simulink model "IEEE_BUS_68_AGC"  (R2025a)
settings: Solver=ode23tb  StartTime=0.0  StopTime=150  FixedStep=Ts  MaxStep=0.0001  RelTol=1e-3
PreLoadFcn:
  | PSSMODEL=1;
  | LPSS=0;
  | WAPSS=0;
  | WAPSS2=0;
  | Ts=50e-5;
InitFcn:
  | PSSMODEL=1;
  | LPSS=0;
  | WAPSS=0;
  | WAPSS2=0;
  | Ts=50e-5;
  | 
  | % Required data to 68 Bus benchmark
  | % clear
  | % clc
  | % Definition for the columns
  | % system base =100 MVA
  | 
  | %% Line data Format (line)
  | % All values are given on the same system base MVA
  | % 1: From bus
  | % 2: To bus
  | % 3: Resistance (pu)
  | % 4: Reactance  (pu)
  | % 5: Charge     (pu)
  | % 6: Transformer Tap Amplitute
  | % 7: base MVA
  | % 8: Nomonal Voltage (KV)
  | 
  | %1   2    3        4       5       6        7      8
  | line=[...
  | 1	54	0	     0.0181	  0	      1.025     100    13.8
  | 2	58	0	     0.025	  0	      1.070     100    13.8
  | 3	62	0	     0.02	  0	      1.070     100    13.8
  | 4	19	0.0007	 0.0142	  0	      1.070     100    13.8
  | 5	20	0.0009	 0.018	  0	      1.009     100    13.8
  | 6	22	0	     0.0143	  0	      1.025     100    13.8
  | 7	23	0.0005	 0.0272	  0	      0         100    13.8
  | 8	25	0.0006	 0.0232	  0	      1.025     100    13.8
  | 9	29	0.0008	 0.0156   0	      1.025     100    13.8
  | 10	31	0	     0.026	  0	      1.04      100    13.8
  | 11	32	0	     0.013	  0	      1.04      100    13.8
  | 12	36	0	     0.0075	  0	      1.04      100    13.8
  | 13	17	0	     0.0033	  0	      1.04      100    13.8
  | 14	41	0	     0.0015	  0	      1         100    13.8
  | 15	42	0	     0.0015	  0	      1         100    13.8
  | 16	18	0	     0.003	  0	      1         100    13.8
  | 17	36	0.0005	 0.0045	  0.32	  0         100    138
  | 17	43	0.0005	 0.0276	  0	      0         100    138
  | 18	42	0.004	 0.06	  2.25    0         100    138
  | 18	49	0.0076	 0.1141	  1.16    0	        100    138
  | 18	50	0.0012	 0.0288	  2.06	  0         100    138
  | 20	19	0.0007	 0.0138	  0       1.06	    100    138
  | 19	68	0.0016	 0.0195	  0.304	  0         100    138
  | 21	22	0.0008	 0.014	  0.2565  0	        100    138
  | 21	68	0.0008	 0.0135	  0.2548  0	        100    138
  | 22	23	0.0006	 0.0096	  0.1846  0	        100    138
  | 23	24	0.0022	 0.035	  0.361	  0         100    138
  | 24	68	0.0003	 0.0059	  0.068	  0         100    138
  | 25	26	0.0032	 0.0323	  0.531	  0         100    138
  | 25	54	0.007	 0.0086	  0.146	  0         100    138
  | 26	27	0.0014	 0.0147	  0.2396  0	        100    138
  | 26	28	0.0043	 0.0474	  0.7802  0	        100    138
  | 26	29	0.0057	 0.0625	  1.029	  0         100    138
  | 27	37	0.0013	 0.0173	  0.3216  0	        100    138
  | 27	53	0.032	 0.32	  0.41	  0         100    138
  | ... (+206 lines)
undefined symbols (not defined in the file or in its folder): D1, Delta
libraries: spsPMUPLLBasedPositiveSequenceLib x90, spsRMSLib x73, spsThreePhaseVIMeasurementLib x69, spsLoadFlowBusLib x69, spsThreePhasePISectionLineLib x64, spsThreePhaseParallelRLCLoadLib x35, spsGenericPowerSystemStabilizerLib x32, spsThreePhaseSeriesRLCLoadLib x21, spsThreePhaseTransformerTwoWindingsLib x21, spsSynchronousMachinepuStandardLib x20, spsExcitationSystemLib x16, spsMultiBandPowerSystemStabilizerLib x16
(part 5 of 8)

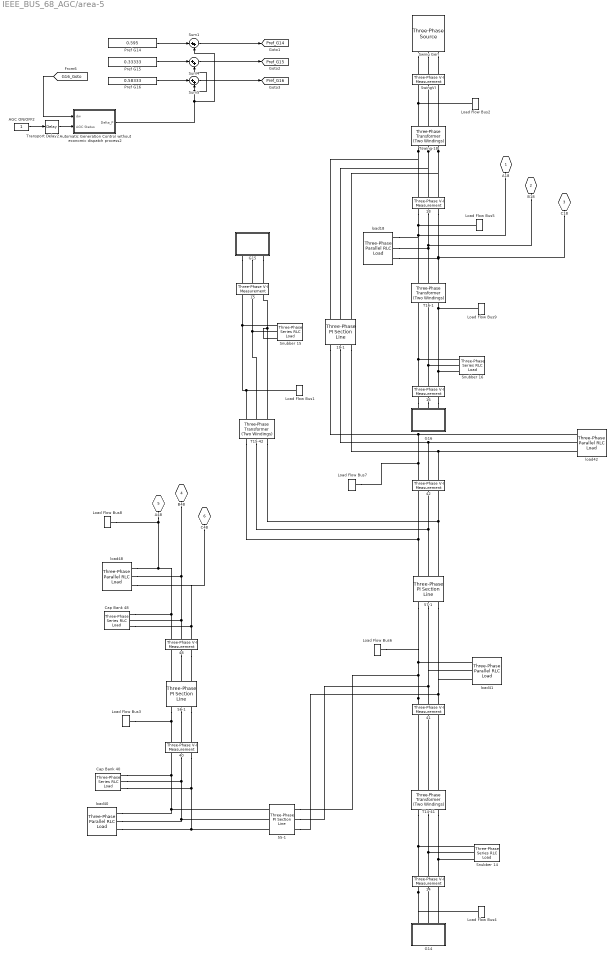
== system IEEE_BUS_68_AGC/area-5 ==
  14 : spsThreePhaseVIMeasurementLib/Three-Phase V-I Measurement  VoltageMeasurement=phase-to-phase  SetLabelV=on  LabelV=Vabc_14  Vpu=off  VpuLL=on  CurrentMeasurement=no  SetLabelI=off  LabelI=Iabc  Ipu=off  Pbase=100e6  Vbase=13.8e3  OutputType=Complex  PhasorSimulation=off  PSBequivalent=0
  15 : spsThreePhaseVIMeasurementLib/Three-Phase V-I Measurement  VoltageMeasurement=phase-to-phase  SetLabelV=on  LabelV=Vabc_15  Vpu=off  VpuLL=on  CurrentMeasurement=no  SetLabelI=off  LabelI=Iabc  Ipu=off  Pbase=100e6  Vbase=13.8e3  OutputType=Complex  PhasorSimulation=off  PSBequivalent=0
  16 : spsThreePhaseVIMeasurementLib/Three-Phase V-I Measurement  VoltageMeasurement=phase-to-phase  SetLabelV=on  LabelV=Vabc_16  Vpu=off  VpuLL=on  CurrentMeasurement=no  SetLabelI=off  LabelI=Iabc  Ipu=off  Pbase=100e6  Vbase=13.8e3  OutputType=Complex  PhasorSimulation=off  PSBequivalent=0
  18 : spsThreePhaseVIMeasurementLib/Three-Phase V-I Measurement  VoltageMeasurement=phase-to-phase  SetLabelV=on  LabelV=Vabc_18  Vpu=off  VpuLL=on  CurrentMeasurement=no  SetLabelI=off  LabelI=Iabc  Ipu=off  Pbase=100e6  Vbase=Bus(18,2)*1e3  OutputType=Complex  PhasorSimulation=off  PSBequivalent=0
  19-1 : spsThreePhasePISectionLineLib/Three-Phase PI Section Line  LConnTagsString=a|b|c  RConnTagsString=A|B|C  Length=1  Frequency=60  Resistances=[line(19,3) 3*line(19,3)]  Inductances=[line(19,4) 3*line(19,4)]  Capacitances=[line(19,5) line(19,5)/3]
  40 : spsThreePhaseVIMeasurementLib/Three-Phase V-I Measurement  VoltageMeasurement=phase-to-phase  SetLabelV=on  LabelV=Vabc_40  Vpu=off  VpuLL=on  CurrentMeasurement=no  SetLabelI=off  LabelI=Iabc  Ipu=off  Pbase=100e6  Vbase=Bus(40,2)*1e3  OutputType=Complex  PhasorSimulation=off  PSBequivalent=0
  41 : spsThreePhaseVIMeasurementLib/Three-Phase V-I Measurement  VoltageMeasurement=phase-to-phase  SetLabelV=on  LabelV=Vabc_41  Vpu=off  VpuLL=on  CurrentMeasurement=no  SetLabelI=off  LabelI=Iabc  Ipu=off  Pbase=100e6  Vbase=Bus(41,2)*1e3  OutputType=Complex  PhasorSimulation=off  PSBequivalent=0
  42 : spsThreePhaseVIMeasurementLib/Three-Phase V-I Measurement  VoltageMeasurement=phase-to-phase  SetLabelV=on  LabelV=Vabc_42  Vpu=off  VpuLL=on  CurrentMeasurement=no  SetLabelI=off  LabelI=Iabc  Ipu=off  Pbase=100e6  Vbase=Bus(42,2)*1e3  OutputType=Complex  PhasorSimulation=off  PSBequivalent=0
  48 : spsThreePhaseVIMeasurementLib/Three-Phase V-I Measurement  VoltageMeasurement=phase-to-phase  SetLabelV=on  LabelV=Vabc_48  Vpu=off  VpuLL=on  CurrentMeasurement=no  SetLabelI=off  LabelI=Iabc  Ipu=off  Pbase=100e6  Vbase=Bus(48,2)*1e3  OutputType=Complex  PhasorSimulation=off  PSBequivalent=0
  55-1 : spsThreePhasePISectionLineLib/Three-Phase PI Section Line  LConnTagsString=a|b|c  RConnTagsString=A|B|C  Length=1  Frequency=60  Resistances=[line(55,3) 3*line(55,3)]  Inductances=[line(55,4) 3*line(55,4)]  Capacitances=[line(55,5) line(55,5)/3]
  56-1 : spsThreePhasePISectionLineLib/Three-Phase PI Section Line  LConnTagsString=a|b|c  RConnTagsString=A|B|C  Length=1  Frequency=60  Resistances=[line(56,3) 3*line(56,3)]  Inductances=[line(56,4) 3*line(56,4)]  Capacitances=[line(56,5) line(56,5)/3]
  57-1 : spsThreePhasePISectionLineLib/Three-Phase PI Section Line  LConnTagsString=a|b|c  RConnTagsString=A|B|C  Length=1  Frequency=60  Resistances=[line(57,3) 3*line(57,3)]  Inductances=[line(57,4) 3*line(57,4)]  Capacitances=[line(57,5) line(57,5)/3]
  AGC ON/OFF2 : Constant
  Automatic Generation Control without economic dispatch process2 : Subsystem
  Cap Bank 40 : spsThreePhaseSeriesRLCLoadLib/Three-Phase Series RLC Load  LConnTagsString=A|B|C  Configuration=Y (grounded)  NominalVoltage=138000  Vabc=[1e3 1e3 1e3]  Vabcp=[1e3 1e3 1e3]  NominalFrequency=60  UnbalancedPower=off  ActivePower=0  InductivePower=0  CapacitivePower=25000000  Pabc=[10e3 9e3 11e3]  QLabc=[100 90 110]  QCabc=[100 90 110]  Pabcp=[10e3 9e3 11e3]  QLabcp=[100 90 110]  QCabcp=[100 90 110]  Measurements=None  LoadType=constant Z
  Cap Bank 48 : spsThreePhaseSeriesRLCLoadLib/Three-Phase Series RLC Load  LConnTagsString=A|B|C  Configuration=Y (grounded)  NominalVoltage=138000  Vabc=[1e3 1e3 1e3]  Vabcp=[1e3 1e3 1e3]  NominalFrequency=60  UnbalancedPower=off  ActivePower=0  InductivePower=0  CapacitivePower=48000000  Pabc=[10e3 9e3 11e3]  QLabc=[100 90 110]  QCabc=[100 90 110]  Pabcp=[10e3 9e3 11e3]  QLabcp=[100 90 110]  QCabcp=[100 90 110]  Measurements=None  LoadType=constant Z
  G14 : Subsystem
  G15 : Subsystem
  G16 : Subsystem
  Load Flow Bus1 : spsLoadFlowBusLib/Load Flow Bus  LConnTagsString=a  Phases=single  Connectors=on one side  ID=BUS_15  Vbase=13.8e3  Vref=1  Vangle=0  VLF=1  VLFb=1  VLFc=1  angleLF=2.569  angleLFb=0  angleLFc=0
  Load Flow Bus2 : spsLoadFlowBusLib/Load Flow Bus  LConnTagsString=a  Phases=single  Connectors=on one side  ID=BUS_Swing  Vbase=13.8e3  Vref=1  Vangle=0  VLF=1  VLFb=1  VLFc=1  angleLF=0  angleLFb=0  angleLFc=0
  Load Flow Bus3 : spsLoadFlowBusLib/Load Flow Bus  LConnTagsString=a  Phases=single  Connectors=on one side  ID=BUS_40  Vbase=138e3  Vref=1  Vangle=0  VLF=1.039  VLFb=1  VLFc=1  angleLF=12.2  angleLFb=0  angleLFc=0
  Load Flow Bus4 : spsLoadFlowBusLib/Load Flow Bus  LConnTagsString=a  Phases=single  Connectors=on one side  ID=BUS_14  Vbase=13.8e3  Vref=1  Vangle=0  VLF=1  VLFb=1  VLFc=1  angleLF=10.16  angleLFb=0  angleLFc=0
  Load Flow Bus5 : spsLoadFlowBusLib/Load Flow Bus  LConnTagsString=a  Phases=single  Connectors=on one side  ID=BUS_18  Vbase=138e3  Vref=1  Vangle=0  VLF=0.9975  VLFb=1  VLFc=1  angleLF=29.96  angleLFb=0  angleLFc=0
  Load Flow Bus6 : spsLoadFlowBusLib/Load Flow Bus  LConnTagsString=a  Phases=single  Connectors=on one side  ID=BUS_41  Vbase=138e3  Vref=1  Vangle=0  VLF=0.9993  VLFb=1  VLFc=1  angleLF=38.63  angleLFb=0  angleLFc=0
  Load Flow Bus7 : spsLoadFlowBusLib/Load Flow Bus  LConnTagsString=a  Phases=single  Connectors=on one side  ID=BUS_42  Vbase=138e3  Vref=1  Vangle=0  VLF=0.9992  VLFb=1  VLFc=1  angleLF=31.71  angleLFb=0  angleLFc=0
  Load Flow Bus8 : spsLoadFlowBusLib/Load Flow Bus  LConnTagsString=a  Phases=single  Connectors=on one side  ID=BUS_48  Vbase=138e3  Vref=1  Vangle=0  VLF=1.031  VLFb=1  VLFc=1  angleLF=6.428  angleLFb=0  angleLFc=0
  Load Flow Bus9 : spsLoadFlowBusLib/Load Flow Bus  LConnTagsString=a  Phases=single  Connectors=on one side  ID=BUS_16  Vbase=13.8e3  Vref=1  Vangle=0  VLF=1  VLFb=1  VLFc=1  angleLF=6  angleLFb=0  angleLFc=0
  Pref G14 : Constant  Value=0.595
  Pref G15 : Constant  Value=0.33333
  Pref G16 : Constant  Value=0.58333
  Snubber 14 : spsThreePhaseSeriesRLCLoadLib/Three-Phase Series RLC Load  LConnTagsString=A|B|C  Configuration=Y (grounded)  NominalVoltage=13.8e3  Vabc=[1e3 1e3 1e3]  Vabcp=[1e3 1e3 1e3]  NominalFrequency=60  UnbalancedPower=off  ActivePower=1000000  InductivePower=0  CapacitivePower=10000000  Pabc=[10e3 9e3 11e3]  QLabc=[100 90 110]  QCabc=[100 90 110]  Pabcp=[10e3 9e3 11e3]  QLabcp=[100 90 110]  QCabcp=[100 90 110]  Measurements=None  LoadType=constant Z
  Snubber 15 : spsThreePhaseSeriesRLCLoadLib/Three-Phase Series RLC Load  LConnTagsString=A|B|C  Configuration=Y (grounded)  NominalVoltage=13.8e3  Vabc=[1e3 1e3 1e3]  Vabcp=[1e3 1e3 1e3]  NominalFrequency=60  UnbalancedPower=off  ActivePower=1000000  InductivePower=0  CapacitivePower=10000000  Pabc=[10e3 9e3 11e3]  QLabc=[100 90 110]  QCabc=[100 90 110]  Pabcp=[10e3 9e3 11e3]  QLabcp=[100 90 110]  QCabcp=[100 90 110]  Measurements=None  LoadType=constant Z
  Snubber 16 : spsThreePhaseSeriesRLCLoadLib/Three-Phase Series RLC Load  LConnTagsString=A|B|C  Configuration=Y (grounded)  NominalVoltage=13.8e3  Vabc=[1e3 1e3 1e3]  Vabcp=[1e3 1e3 1e3]  NominalFrequency=60  UnbalancedPower=off  ActivePower=1000000  InductivePower=0  CapacitivePower=10000000  Pabc=[10e3 9e3 11e3]  QLabc=[100 90 110]  QCabc=[100 90 110]  Pabcp=[10e3 9e3 11e3]  QLabcp=[100 90 110]  QCabcp=[100 90 110]  Measurements=None  LoadType=constant Z
  Sum1 : Sum  Inputs=|++
  Sum4 : Sum  Inputs=|++
  Sum5 : Sum  Inputs=|++
  Swing Gen : spsThreePhaseSourceLib/Three-Phase Source  InternalConnection=Yg  VoltagePhases=off  Voltage=(13800)*1.02429  PhaseAngle=0.1743  Voltage_phases=[25e3 25e3 25e3]/sqrt(3)  PhaseAngles_phases=[0 -120 +120]  Frequency=60  NonIdealSource=on  SpecifyImpedance=on  Resistance=0.8929  Inductance=16.58e-3  ShortCircuitLevel=3600e6  BaseVoltage=13.8e3  XRratio=7  BusType=swing  Pref=1000000000  Qref=0  Prefabc=[10e3, 10e3, 10e3]  Qrefabc=[0, 0, 0]  Qmin=-Inf  Qmax=Inf
  SwingVI : spsThreePhaseVIMeasurementLib/Three-Phase V-I Measurement  VoltageMeasurement=phase-to-phase  SetLabelV=on  LabelV=Vabc_Swing  Vpu=off  VpuLL=on  CurrentMeasurement=no  SetLabelI=off  LabelI=Iabc  Ipu=off  Pbase=100e6  Vbase=13.8e3  OutputType=Complex  PhasorSimulation=off  PSBequivalent=0
  T14-41 : spsThreePhaseTransformerTwoWindingsLib/Three-Phase Transformer (Two Windings)  Winding1Connection=Delta (D1)  Winding2Connection=Yg  CoreType=Three single-phase transformers  SetSaturation=off  Hysteresis=off  DataFile='hysteresis'  SetInitialFlux=off  Measurements=None  UNITS=pu  NominalPower=[ 100e6 , 60 ]  Winding1=[ 13.8e3 , 0.0 , 0 ]  Winding2=[ 138e3 , 0.0 , 0.0015 ]  Rm=500  Lm=500  L0=0.5  Saturation=[ 0,0 ; 0.0024,1.2 ; 1.0,1.52 ]  InitialFluxes=[ 0.8 , -0.8 , 0.7 ]  BreakLoop=off  DiscreteSolver=Trapezoidal robust  DataType=off  TransfoNumber=1
  T15-42 : spsThreePhaseTransformerTwoWindingsLib/Three-Phase Transformer (Two Windings)  Winding1Connection=Delta (D1)  Winding2Connection=Yg  CoreType=Three single-phase transformers  SetSaturation=off  Hysteresis=off  DataFile='hysteresis'  SetInitialFlux=off  Measurements=None  UNITS=pu  NominalPower=[ 100e6 , 60 ]  Winding1=[ 13.8e3 , 0.0 , 0 ]  Winding2=[ 138e3 , 0.0, 0.0015 ]  Rm=500  Lm=500  L0=0.5  Saturation=[ 0,0 ; 0.0024,1.2 ; 1.0,1.52 ]  InitialFluxes=[ 0.8 , -0.8 , 0.7 ]  BreakLoop=off  DiscreteSolver=Trapezoidal robust  DataType=off  TransfoNumber=1
  T16-1 : spsThreePhaseTransformerTwoWindingsLib/Three-Phase Transformer (Two Windings)  Winding1Connection=Delta (D1)  Winding2Connection=Yg  CoreType=Three single-phase transformers  SetSaturation=off  Hysteresis=off  DataFile='hysteresis'  SetInitialFlux=off  Measurements=None  UNITS=pu  NominalPower=[ 100e6 , 60 ]  Winding1=[ 13.8e3 , 0.0 , 0 ]  Winding2=[ 138e3 , 0.0, 0.003 ]  Rm=500  Lm=500  L0=0.5  Saturation=[ 0,0 ; 0.0024,1.2 ; 1.0,1.52 ]  InitialFluxes=[ 0.8 , -0.8 , 0.7 ]  BreakLoop=off  DiscreteSolver=Trapezoidal robust  DataType=off  TransfoNumber=1
  Transport Delay2 : TransportDelay  DelayTime=20
  Tswing-18 : spsThreePhaseTransformerTwoWindingsLib/Three-Phase Transformer (Two Windings)  Winding1Connection=Delta (D1)  Winding2Connection=Yg  CoreType=Three single-phase transformers  SetSaturation=off  Hysteresis=off  DataFile='hysteresis'  SetInitialFlux=off  Measurements=None  UNITS=pu  NominalPower=[ 100e6 , 60 ]  Winding1=[ 13.8e3 , 0.0 , 0 ]  Winding2=[ 138e3 , 0.0, 0.003 ]  Rm=500  Lm=500  L0=0.5  Saturation=[ 0,0 ; 0.0024,1.2 ; 1.0,1.52 ]  InitialFluxes=[ 0.8 , -0.8 , 0.7 ]  BreakLoop=off  DiscreteSolver=Trapezoidal robust  DataType=off  TransfoNumber=1
  load18 : spsThreePhaseParallelRLCLoadLib/Three-Phase Parallel RLC Load  LConnTagsString=A|B|C  Configuration=Y (grounded)  NominalVoltage=(138000)*0.997483  Vabc=[1e3 1e3 1e3]  Vabcp=[1e3 1e3 1e3]  NominalFrequency=60  UnbalancedPower=off  ActivePower=2211000000  InductivePower=123000000  CapacitivePower=0  Pabc=[10e3 9e3 11e3]  QLabc=[100 90 110]  QCabc=[100 90 110]  Pabcp=[10e3 9e3 11e3]  QLabcp=[100 90 110]  QCabcp=[100 90 110]  Measurements=None  LoadType=constant PQ
  load40 : spsThreePhaseParallelRLCLoadLib/Three-Phase Parallel RLC Load  LConnTagsString=A|B|C  Configuration=Y (grounded)  NominalVoltage=(138000)*1.03949  Vabc=[1e3 1e3 1e3]  Vabcp=[1e3 1e3 1e3]  NominalFrequency=60  UnbalancedPower=off  ActivePower=66000000  InductivePower=24000000  CapacitivePower=0  Pabc=[10e3 9e3 11e3]  QLabc=[100 90 110]  QCabc=[100 90 110]  Pabcp=[10e3 9e3 11e3]  QLabcp=[100 90 110]  QCabcp=[100 90 110]  Measurements=None  LoadType=constant PQ
  load41 : spsThreePhaseParallelRLCLoadLib/Three-Phase Parallel RLC Load  LConnTagsString=A|B|C  Configuration=Y (grounded)  NominalVoltage=(138000)*0.999333  Vabc=[1e3 1e3 1e3]  Vabcp=[1e3 1e3 1e3]  NominalFrequency=60  UnbalancedPower=off  ActivePower=1000000000  InductivePower=250000000  CapacitivePower=0  Pabc=[10e3 9e3 11e3]  QLabc=[100 90 110]  QCabc=[100 90 110]  Pabcp=[10e3 9e3 11e3]  QLabcp=[100 90 110]  QCabcp=[100 90 110]  Measurements=None  LoadType=constant PQ
  load42 : spsThreePhaseParallelRLCLoadLib/Three-Phase Parallel RLC Load  LConnTagsString=A|B|C  Configuration=Y (grounded)  NominalVoltage=(138000)*0.99916  Vabc=[1e3 1e3 1e3]  Vabcp=[1e3 1e3 1e3]  NominalFrequency=60  UnbalancedPower=off  ActivePower=1150000000  InductivePower=250000000  CapacitivePower=0  Pabc=[10e3 9e3 11e3]  QLabc=[100 90 110]  QCabc=[100 90 110]  Pabcp=[10e3 9e3 11e3]  QLabcp=[100 90 110]  QCabcp=[100 90 110]  Measurements=None  LoadType=constant PQ
  load48 : spsThreePhaseParallelRLCLoadLib/Three-Phase Parallel RLC Load  LConnTagsString=A|B|C  Configuration=Y (grounded)  NominalVoltage=(138000)*1.03085  Vabc=[1e3 1e3 1e3]  Vabcp=[1e3 1e3 1e3]  NominalFrequency=60  UnbalancedPower=off  ActivePower=500000000  InductivePower=101500000  CapacitivePower=0  Pabc=[10e3 9e3 11e3]  QLabc=[100 90 110]  QCabc=[100 90 110]  Pabcp=[10e3 9e3 11e3]  QLabcp=[100 90 110]  QCabcp=[100 90 110]  Measurements=None  LoadType=constant PQ
  A18 : PMIOPort  Tag=PMCPort  Side=Right
  B18 : PMIOPort  Tag=PMCPort  Port=2  Side=Right
  C18 : PMIOPort  Tag=PMCPort  Port=3  Side=Right
  B48 : PMIOPort  Tag=PMCPort  Port=4  Side=Right
  A48 : PMIOPort  Tag=PMCPort  Port=5  Side=Right
  C48 : PMIOPort  Tag=PMCPort  Port=6  Side=Right
  tag scope: Pref_G14=global, Pref_G15=global, Pref_G16=global
  wires:
  Sum1/1 -> [Pref_G14]
  Pref G15/1 -> Sum4/1
  Sum5/1 -> [Pref_G16]
  Automatic Generation Control without economic dispatch process2/1(Delta_P) -> Sum1/2, Sum4/2, Sum5/2
  Sum4/1 -> [Pref_G15]
  Pref G14/1 -> Sum1/1
  Pref G16/1 -> Sum5/1
  [G16_Goto] -> Automatic Generation Control without economic dispatch process2/1(dw)
  AGC ON/OFF2/1 -> Transport Delay2/1
  Transport Delay2/1 -> Automatic Generation Control without economic dispatch process2/2(AGC Status)
  connections:
  T14-41/LConn3 -- 14/LConn3 -- Snubber 14/LConn3
  T14-41/LConn2 -- Snubber 14/LConn2 -- 14/LConn2
  18/LConn1 -- Load Flow Bus5/LConn1 -- load18/LConn1 -- T16-1/RConn1 -- A18/RConn1
  Tswing-18/LConn2 -- SwingVI/LConn2
  T15-42/LConn3 -- Snubber 15/LConn3 -- 15/LConn3
  19-1/RConn1 -- load42/LConn1 -- 42/LConn1 -- Load Flow Bus7/LConn1
  Tswing-18/LConn3 -- SwingVI/LConn3
  load18/LConn3 -- 18/LConn3 -- C18/RConn1 -- T16-1/RConn3
  48/RConn2 -- 56-1/LConn2
  T14-41/RConn1 -- 41/RConn1
  Swing Gen/RConn3 -- SwingVI/RConn3
  T15-42/LConn2 -- Snubber 15/LConn2 -- 15/LConn2
  56-1/RConn3 -- 40/LConn3
  57-1/RConn2 -- load41/LConn2 -- 55-1/RConn2 -- 41/LConn2
  T14-41/RConn3 -- 41/RConn3
  T14-41/LConn1 -- Snubber 14/LConn1 -- 14/LConn1
  Tswing-18/RConn1 -- 18/RConn1 -- 19-1/LConn1
  56-1/RConn1 -- 40/LConn1 -- Load Flow Bus3/LConn1
  56-1/RConn2 -- 40/LConn2
  T15-42/LConn1 -- Load Flow Bus1/LConn1 -- Snubber 15/LConn1 -- 15/LConn1
  G15/LConn1 -- 15/RConn1
  Swing Gen/RConn1 -- SwingVI/RConn1
  Tswing-18/LConn1 -- Load Flow Bus2/LConn1 -- SwingVI/LConn1
  55-1/LConn1 -- load40/LConn1 -- 40/RConn1 -- Cap Bank 40/LConn1
  load18/LConn2 -- T16-1/RConn2 -- 18/LConn2 -- B18/RConn1
  Tswing-18/RConn3 -- 18/RConn3 -- 19-1/LConn3
  41/LConn1 -- Load Flow Bus6/LConn1 -- 57-1/RConn1 -- load41/LConn1 -- 55-1/RConn1
  14/RConn1 -- Load Flow Bus4/LConn1 -- G14/LConn1
  G15/LConn3 -- 15/RConn3
  Tswing-18/RConn2 -- 18/RConn2 -- 19-1/LConn2
  G14/LConn3 -- 14/RConn3
  56-1/LConn1 -- 48/RConn1
  G15/LConn2 -- 15/RConn2
  T15-42/RConn2 -- 42/RConn2 -- 57-1/LConn2
  57-1/RConn3 -- load41/LConn3 -- 55-1/RConn3 -- 41/LConn3
  48/RConn3 -- 56-1/LConn3
  T15-42/RConn1 -- 42/RConn1 -- 57-1/LConn1
  40/RConn2 -- load40/LConn2 -- 55-1/LConn2 -- Cap Bank 40/LConn2
  load48/LConn3 -- C48/RConn1 -- Cap Bank 48/LConn3 -- 48/LConn3
  G14/LConn2 -- 14/RConn2
  T15-42/RConn3 -- 42/RConn3 -- 57-1/LConn3
  Swing Gen/RConn2 -- SwingVI/RConn2
  40/RConn3 -- load40/LConn3 -- 55-1/LConn3 -- Cap Bank 40/LConn3
  A48/RConn1 -- load48/LConn1 -- Cap Bank 48/LConn1 -- 48/LConn1 -- Load Flow Bus8/LConn1
  load48/LConn2 -- Cap Bank 48/LConn2 -- 48/LConn2 -- B48/RConn1
  T14-41/RConn2 -- 41/RConn2
  Snubber 16/LConn1 -- 16/LConn1 -- T16-1/LConn1
  Snubber 16/LConn2 -- 16/LConn2 -- T16-1/LConn2
  Snubber 16/LConn3 -- 16/LConn3 -- Load Flow Bus9/LConn1 -- T16-1/LConn3
  16/RConn1 -- G16/LConn1
  16/RConn2 -- G16/LConn2
  16/RConn3 -- G16/LConn3
  19-1/RConn2 -- load42/LConn2 -- 42/LConn2
  19-1/RConn3 -- load42/LConn3 -- 42/LConn3

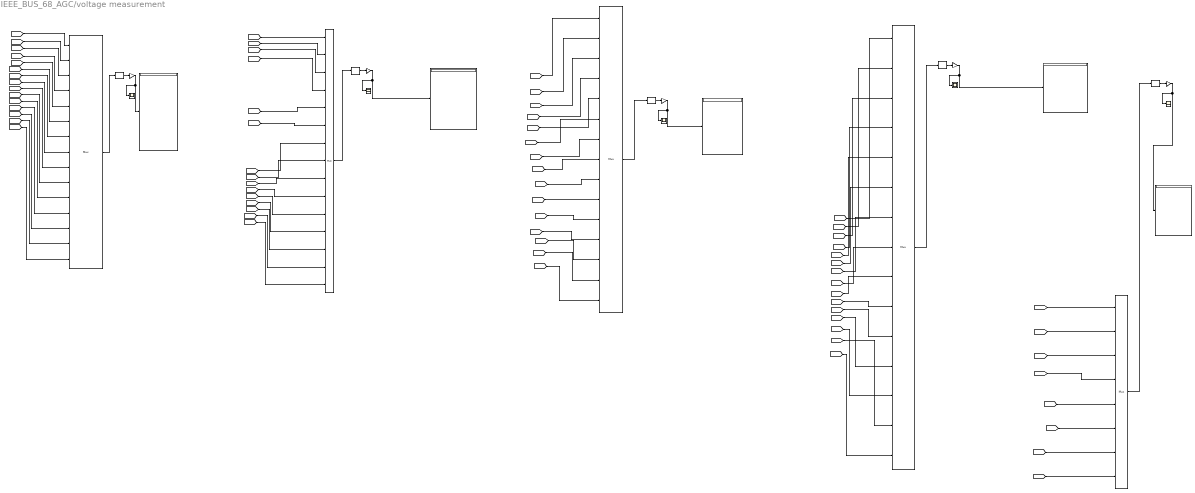
== system IEEE_BUS_68_AGC/voltage measurement  ==
  Display{,1..4} (5 alike) : Display
  Gain{1..4} (4 alike) : Gain  Gain=2*sqrt(2)/sqrt(3)
  Gain5 : Gain  Gain=2/sqrt(3)
  Mux{1..4} (4 alike) : Mux  Inputs=15
  Mux5 : Mux  Inputs=8
  RMS{1..5} (5 alike) : spsRMSLib/RMS  TrueRMS=on  Freq=60  RMSInit=120  Ts=Ts
  Scope{1..5} (5 alike) : Scope
      Scope1 settings: ActiveDisplayYMinimum=1.1040754894439568  ActiveDisplayYMaximum=1.2513201627894044
      Scope2 settings: ActiveDisplayYMinimum=1.0150637311703361  ActiveDisplayYMaximum=1.3487833140208574
      Scope3 settings: ActiveDisplayYMinimum=0.86021415644856791  ActiveDisplayYMaximum=1.7941077878421252  DataLoggingVariableName=ScopeData2
      Scope4 settings: ActiveDisplayYMinimum=-3  ActiveDisplayYMaximum=3  DataLoggingVariableName=ScopeData3
      Scope5 settings: ActiveDisplayYMinimum=-3  ActiveDisplayYMaximum=3  DataLoggingVariableName=ScopeData4
  wires:
  Mux1/1 -> RMS2/1
  [Vabc_05] -> Mux1/5
  [Vabc_06] -> Mux1/6
  Gain2/1 -> Display/1, Scope1/1
  [Vabc_03] -> Mux1/3
  [Vabc_11] -> Mux1/11
  [Vabc_10] -> Mux1/10
  [Vabc_07] -> Mux1/7
  [Vabc_09] -> Mux1/9
  [Vabc_01] -> Mux1/1
  [Vabc_13] -> Mux1/13
  [Vabc_02] -> Mux1/2
  [Vabc_12] -> Mux1/12
  [Vabc_14] -> Mux1/14
  [Vabc_08] -> Mux1/8
  RMS2/1 -> Gain2/1
  [Vabc_04] -> Mux1/4
  [Vabc_15] -> Mux1/15
  Mux2/1 -> RMS1/1
  RMS1/1 -> Gain1/1
  Gain1/1 -> Scope2/1, Display1/1
  [Vabc_16] -> Mux2/1
  [Vabc_17] -> Mux2/2
  [Vabc_18] -> Mux2/3
  Gain3/1 -> Scope3/1, Display2/1
  RMS3/1 -> Gain3/1
  Mux3/1 -> RMS3/1
  Gain4/1 -> Scope4/1, Display3/1
  RMS4/1 -> Gain4/1
  Mux4/1 -> RMS4/1
  [Vabc_19] -> Mux2/4
  [Vabc_20] -> Mux2/5
  [Vabc_21] -> Mux2/6
  [Vabc_22] -> Mux2/7
  [Vabc_23] -> Mux2/8
  [Vabc_24] -> Mux2/9
  [Vabc_25] -> Mux2/10
  [Vabc_26] -> Mux2/11
  [Vabc_27] -> Mux2/12
  [Vabc_28] -> Mux2/13
  [Vabc_29] -> Mux2/14
  [Vabc_30] -> Mux2/15
  [Vabc_31] -> Mux3/1
  [Vabc_32] -> Mux3/2
  [Vabc_33] -> Mux3/3
  [Vabc_34] -> Mux3/4
  [Vabc_35] -> Mux3/5
  [Vabc_36] -> Mux3/6
  [Vabc_37] -> Mux3/7
  [Vabc_38] -> Mux3/8
  [Vabc_39] -> Mux3/9
  [Vabc_40] -> Mux3/10
  [Vabc_41] -> Mux3/11
  [Vabc_42] -> Mux3/12
  [Vabc_43] -> Mux3/13
  [Vabc_44] -> Mux3/14
  [Vabc_45] -> Mux3/15
  [Vabc_46] -> Mux4/1
  [Vabc_47] -> Mux4/2
  [Vabc_48] -> Mux4/3
  [Vabc_49] -> Mux4/4
  [Vabc_50] -> Mux4/5
  [Vabc_51] -> Mux4/6
  [Vabc_52] -> Mux4/7
  [Vabc_53] -> Mux4/8
  [Vabc_54] -> Mux4/9
  [Vabc_55] -> Mux4/10
  [Vabc_56] -> Mux4/11
  [Vabc_57] -> Mux4/12
  [Vabc_58] -> Mux4/13
  [Vabc_59] -> Mux4/14
  [Vabc_60] -> Mux4/15
  Gain5/1 -> Display4/1, Scope5/1
  RMS5/1 -> Gain5/1
  Mux5/1 -> RMS5/1
  [Vabc_61] -> Mux5/1
  [Vabc_62] -> Mux5/2
  [Vabc_63] -> Mux5/3
  [Vabc_64] -> Mux5/4
  [Vabc_65] -> Mux5/5
  [Vabc_66] -> Mux5/6
  [Vabc_67] -> Mux5/7
  [Vabc_68] -> Mux5/8

== system IEEE_BUS_68_AGC/Monitoring/area1 ==
  K_04 : Gain  Gain=sqrt(2)
  K_05 : Gain  Gain=sqrt(2)
  K_06 : Gain  Gain=sqrt(2)
  K_07 : Gain  Gain=sqrt(2)
  K_{19..24,68} (7 alike) : Gain  Gain=sqrt(2)
  Log_V_area1 : ToWorkspace  VariableName=V_area1  SaveFormat=Structure With Time  SampleTime=0.00833333333333333
  MuxV : Mux  Inputs=11
  RMS_04 : spsRMSLib/RMS  TrueRMS=on  Freq=60  RMSInit=120  Ts=Ts
  RMS_05 : spsRMSLib/RMS  TrueRMS=on  Freq=60  RMSInit=120  Ts=Ts
  RMS_06 : spsRMSLib/RMS  TrueRMS=on  Freq=60  RMSInit=120  Ts=Ts
  RMS_07 : spsRMSLib/RMS  TrueRMS=on  Freq=60  RMSInit=120  Ts=Ts
  RMS_{19..24,68} (7 alike) : spsRMSLib/RMS  TrueRMS=on  Freq=60  RMSInit=120  Ts=Ts
  Scope_V_area1 : Scope
      settings: ActiveDisplayYMinimum=0.97001723692271469  ActiveDisplayYMaximum=1.0992415688687989
  wires:
  [Vabc_04] -> RMS_04/1
  RMS_04/1 -> K_04/1
  [Vabc_05] -> RMS_05/1
  RMS_05/1 -> K_05/1
  [Vabc_06] -> RMS_06/1
  RMS_06/1 -> K_06/1
  [Vabc_07] -> RMS_07/1
  RMS_07/1 -> K_07/1
  [Vabc_19] -> RMS_19/1
  RMS_19/1 -> K_19/1
  [Vabc_20] -> RMS_20/1
  RMS_20/1 -> K_20/1
  [Vabc_21] -> RMS_21/1
  RMS_21/1 -> K_21/1
  [Vabc_22] -> RMS_22/1
  RMS_22/1 -> K_22/1
  [Vabc_23] -> RMS_23/1
  RMS_23/1 -> K_23/1
  [Vabc_24] -> RMS_24/1
  RMS_24/1 -> K_24/1
  [Vabc_68] -> RMS_68/1
  RMS_68/1 -> K_68/1
  K_04/1 -> MuxV/1
  K_05/1 -> MuxV/2
  K_06/1 -> MuxV/3
  K_07/1 -> MuxV/4
  K_19/1 -> MuxV/5
  K_20/1 -> MuxV/6
  K_21/1 -> MuxV/7
  K_22/1 -> MuxV/8
  K_23/1 -> MuxV/9
  K_24/1 -> MuxV/10
  K_68/1 -> MuxV/11
  MuxV/1 -> Scope_V_area1/1, Log_V_area1/1

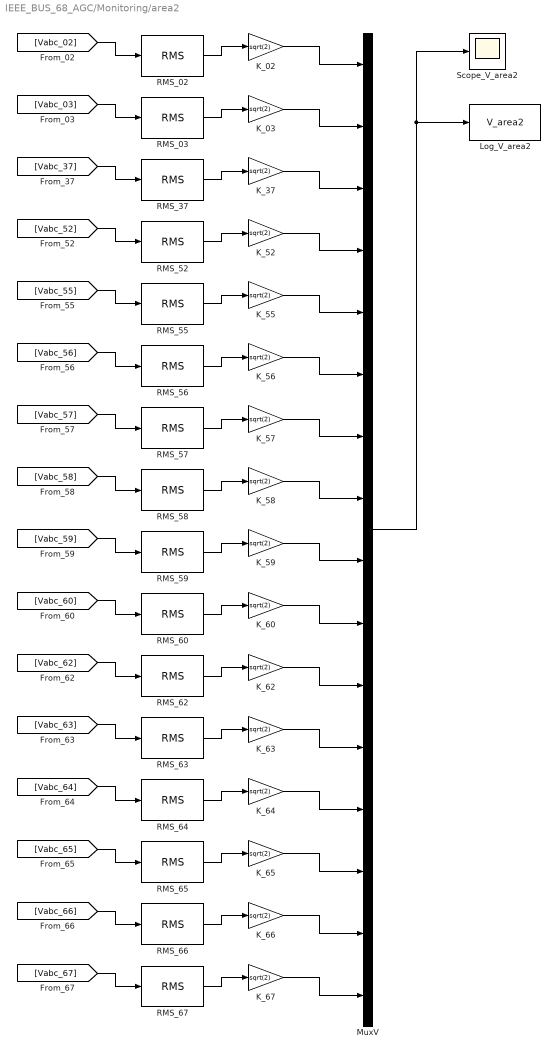
== system IEEE_BUS_68_AGC/Monitoring/area2 ==
  K_02 : Gain  Gain=sqrt(2)
  K_03 : Gain  Gain=sqrt(2)
  K_{37,52,55..60,62..67} (14 alike) : Gain  Gain=sqrt(2)
  Log_V_area2 : ToWorkspace  VariableName=V_area2  SaveFormat=Structure With Time  SampleTime=0.00833333333333333
  MuxV : Mux  Inputs=16
  RMS_02 : spsRMSLib/RMS  TrueRMS=on  Freq=60  RMSInit=120  Ts=Ts
  RMS_03 : spsRMSLib/RMS  TrueRMS=on  Freq=60  RMSInit=120  Ts=Ts
  RMS_{37,52,55..60,62..67} (14 alike) : spsRMSLib/RMS  TrueRMS=on  Freq=60  RMSInit=120  Ts=Ts
  Scope_V_area2 : Scope
      settings: ActiveDisplayYMinimum=0.91572910702674792  ActiveDisplayYMaximum=1.0408509995472783
  wires:
  [Vabc_02] -> RMS_02/1
  RMS_02/1 -> K_02/1
  [Vabc_03] -> RMS_03/1
  RMS_03/1 -> K_03/1
  [Vabc_37] -> RMS_37/1
  RMS_37/1 -> K_37/1
  [Vabc_52] -> RMS_52/1
  RMS_52/1 -> K_52/1
  [Vabc_55] -> RMS_55/1
  RMS_55/1 -> K_55/1
  [Vabc_56] -> RMS_56/1
  RMS_56/1 -> K_56/1
  [Vabc_57] -> RMS_57/1
  RMS_57/1 -> K_57/1
  [Vabc_58] -> RMS_58/1
  RMS_58/1 -> K_58/1
  [Vabc_59] -> RMS_59/1
  RMS_59/1 -> K_59/1
  [Vabc_60] -> RMS_60/1
  RMS_60/1 -> K_60/1
  [Vabc_62] -> RMS_62/1
  RMS_62/1 -> K_62/1
  [Vabc_63] -> RMS_63/1
  RMS_63/1 -> K_63/1
  [Vabc_64] -> RMS_64/1
  RMS_64/1 -> K_64/1
  [Vabc_65] -> RMS_65/1
  RMS_65/1 -> K_65/1
  [Vabc_66] -> RMS_66/1
  RMS_66/1 -> K_66/1
  [Vabc_67] -> RMS_67/1
  RMS_67/1 -> K_67/1
  K_02/1 -> MuxV/1
  K_03/1 -> MuxV/2
  K_37/1 -> MuxV/3
  K_52/1 -> MuxV/4
  K_55/1 -> MuxV/5
  K_56/1 -> MuxV/6
  K_57/1 -> MuxV/7
  K_58/1 -> MuxV/8
  K_59/1 -> MuxV/9
  K_60/1 -> MuxV/10
  K_62/1 -> MuxV/11
  K_63/1 -> MuxV/12
  K_64/1 -> MuxV/13
  K_65/1 -> MuxV/14
  K_66/1 -> MuxV/15
  K_67/1 -> MuxV/16
  MuxV/1 -> Scope_V_area2/1, Log_V_area2/1

== system IEEE_BUS_68_AGC/Monitoring/area3 ==
  K_01 : Gain  Gain=sqrt(2)
  K_08 : Gain  Gain=sqrt(2)
  K_09 : Gain  Gain=sqrt(2)
  K_{25..29,47,53..54} (8 alike) : Gain  Gain=sqrt(2)
  Log_V_area3 : ToWorkspace  VariableName=V_area3  SaveFormat=Structure With Time  SampleTime=0.00833333333333333
  MuxV : Mux  Inputs=11
  RMS_01 : spsRMSLib/RMS  TrueRMS=on  Freq=60  RMSInit=120  Ts=Ts
  RMS_08 : spsRMSLib/RMS  TrueRMS=on  Freq=60  RMSInit=120  Ts=Ts
  RMS_09 : spsRMSLib/RMS  TrueRMS=on  Freq=60  RMSInit=120  Ts=Ts
  RMS_{25..29,47,53..54} (8 alike) : spsRMSLib/RMS  TrueRMS=on  Freq=60  RMSInit=120  Ts=Ts
  Scope_V_area3 : Scope
      settings: ActiveDisplayYMinimum=1.0093611683523231  ActiveDisplayYMaximum=1.0798118485648311
  wires:
  [Vabc_01] -> RMS_01/1
  RMS_01/1 -> K_01/1
  [Vabc_08] -> RMS_08/1
  RMS_08/1 -> K_08/1
  [Vabc_09] -> RMS_09/1
  RMS_09/1 -> K_09/1
  [Vabc_25] -> RMS_25/1
  RMS_25/1 -> K_25/1
  [Vabc_26] -> RMS_26/1
  RMS_26/1 -> K_26/1
  [Vabc_27] -> RMS_27/1
  RMS_27/1 -> K_27/1
  [Vabc_28] -> RMS_28/1
  RMS_28/1 -> K_28/1
  [Vabc_29] -> RMS_29/1
  RMS_29/1 -> K_29/1
  [Vabc_47] -> RMS_47/1
  RMS_47/1 -> K_47/1
  [Vabc_53] -> RMS_53/1
  RMS_53/1 -> K_53/1
  [Vabc_54] -> RMS_54/1
  RMS_54/1 -> K_54/1
  K_01/1 -> MuxV/1
  K_08/1 -> MuxV/2
  K_09/1 -> MuxV/3
  K_25/1 -> MuxV/4
  K_26/1 -> MuxV/5
  K_27/1 -> MuxV/6
  K_28/1 -> MuxV/7
  K_29/1 -> MuxV/8
  K_47/1 -> MuxV/9
  K_53/1 -> MuxV/10
  K_54/1 -> MuxV/11
  MuxV/1 -> Scope_V_area3/1, Log_V_area3/1

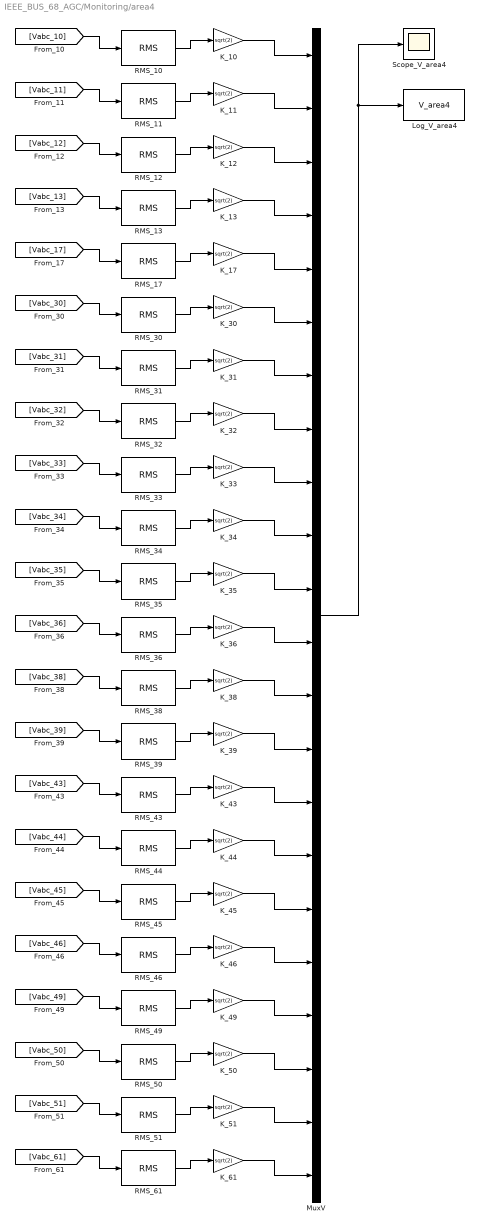
== system IEEE_BUS_68_AGC/Monitoring/area4 ==
  K_{10..13,17,30..36,38..39,43..46,49..51,61} (22 alike) : Gain  Gain=sqrt(2)
  Log_V_area4 : ToWorkspace  VariableName=V_area4  SaveFormat=Structure With Time  SampleTime=0.00833333333333333
  MuxV : Mux  Inputs=22
  RMS_{10..13,17,30..36,38..39,43..46,49..51,61} (22 alike) : spsRMSLib/RMS  TrueRMS=on  Freq=60  RMSInit=120  Ts=Ts
  Scope_V_area4 : Scope
      settings: ActiveDisplayYMinimum=0.96059629199223218  ActiveDisplayYMaximum=1.1592161698878025
  wires:
  [Vabc_10] -> RMS_10/1
  RMS_10/1 -> K_10/1
  [Vabc_11] -> RMS_11/1
  RMS_11/1 -> K_11/1
  [Vabc_12] -> RMS_12/1
  RMS_12/1 -> K_12/1
  [Vabc_13] -> RMS_13/1
  RMS_13/1 -> K_13/1
  [Vabc_17] -> RMS_17/1
  RMS_17/1 -> K_17/1
  [Vabc_30] -> RMS_30/1
  RMS_30/1 -> K_30/1
  [Vabc_31] -> RMS_31/1
  RMS_31/1 -> K_31/1
  [Vabc_32] -> RMS_32/1
  RMS_32/1 -> K_32/1
  [Vabc_33] -> RMS_33/1
  RMS_33/1 -> K_33/1
  [Vabc_34] -> RMS_34/1
  RMS_34/1 -> K_34/1
  [Vabc_35] -> RMS_35/1
  RMS_35/1 -> K_35/1
  [Vabc_36] -> RMS_36/1
  RMS_36/1 -> K_36/1
  [Vabc_38] -> RMS_38/1
  RMS_38/1 -> K_38/1
  [Vabc_39] -> RMS_39/1
  RMS_39/1 -> K_39/1
  [Vabc_43] -> RMS_43/1
  RMS_43/1 -> K_43/1
  [Vabc_44] -> RMS_44/1
  RMS_44/1 -> K_44/1
  [Vabc_45] -> RMS_45/1
  RMS_45/1 -> K_45/1
  [Vabc_46] -> RMS_46/1
  RMS_46/1 -> K_46/1
  [Vabc_49] -> RMS_49/1
  RMS_49/1 -> K_49/1
  [Vabc_50] -> RMS_50/1
  RMS_50/1 -> K_50/1
  [Vabc_51] -> RMS_51/1
  RMS_51/1 -> K_51/1
  [Vabc_61] -> RMS_61/1
  RMS_61/1 -> K_61/1
  K_10/1 -> MuxV/1
  K_11/1 -> MuxV/2
  K_12/1 -> MuxV/3
  K_13/1 -> MuxV/4
  K_17/1 -> MuxV/5
  K_30/1 -> MuxV/6
  K_31/1 -> MuxV/7
  K_32/1 -> MuxV/8
  K_33/1 -> MuxV/9
  K_34/1 -> MuxV/10
  K_35/1 -> MuxV/11
  K_36/1 -> MuxV/12
  K_38/1 -> MuxV/13
  K_39/1 -> MuxV/14
  K_43/1 -> MuxV/15
  K_44/1 -> MuxV/16
  K_45/1 -> MuxV/17
  K_46/1 -> MuxV/18
  K_49/1 -> MuxV/19
  K_50/1 -> MuxV/20
  K_51/1 -> MuxV/21
  K_61/1 -> MuxV/22
  MuxV/1 -> Scope_V_area4/1, Log_V_area4/1

== system IEEE_BUS_68_AGC/Monitoring/area5 ==
  K_{14..16,18,40..42,48} (8 alike) : Gain  Gain=sqrt(2)
  Log_V_area5 : ToWorkspace  VariableName=V_area5  SaveFormat=Structure With Time  SampleTime=0.00833333333333333
  MuxV : Mux  Inputs=8
  RMS_{14..16,18,40..42,48} (8 alike) : spsRMSLib/RMS  TrueRMS=on  Freq=60  RMSInit=120  Ts=Ts
  Scope_V_area5 : Scope
      settings: ActiveDisplayYMinimum=1.0033027494263385  ActiveDisplayYMaximum=1.0540733460084368
  wires:
  [Vabc_14] -> RMS_14/1
  RMS_14/1 -> K_14/1
  [Vabc_15] -> RMS_15/1
  RMS_15/1 -> K_15/1
  [Vabc_16] -> RMS_16/1
  RMS_16/1 -> K_16/1
  [Vabc_18] -> RMS_18/1
  RMS_18/1 -> K_18/1
  [Vabc_40] -> RMS_40/1
  RMS_40/1 -> K_40/1
  [Vabc_41] -> RMS_41/1
  RMS_41/1 -> K_41/1
  [Vabc_42] -> RMS_42/1
  RMS_42/1 -> K_42/1
  [Vabc_48] -> RMS_48/1
  RMS_48/1 -> K_48/1
  K_14/1 -> MuxV/1
  K_15/1 -> MuxV/2
  K_16/1 -> MuxV/3
  K_18/1 -> MuxV/4
  K_40/1 -> MuxV/5
  K_41/1 -> MuxV/6
  K_42/1 -> MuxV/7
  K_48/1 -> MuxV/8
  MuxV/1 -> Scope_V_area5/1, Log_V_area5/1

== system IEEE_BUS_68_AGC/PMU Monitoring/area1 ==
  Log_F_area1 : ToWorkspace  VariableName=F_area1  SaveFormat=Structure With Time  SampleTime=0.00833333333333333
  Log_V_area1 : ToWorkspace  VariableName=V_area1  SaveFormat=Structure With Time  SampleTime=0.00833333333333333
  MuxF : Mux  Inputs=11
  MuxV : Mux  Inputs=11
  PMU_04 : spsPMUPLLBasedPositiveSequenceLib/PMU (PLL-Based, Positive-Sequence)  nominalFrequency=60  samplingRate=24  reportingFactor=1
  PMU_05 : spsPMUPLLBasedPositiveSequenceLib/PMU (PLL-Based, Positive-Sequence)  nominalFrequency=60  samplingRate=24  reportingFactor=1
  PMU_06 : spsPMUPLLBasedPositiveSequenceLib/PMU (PLL-Based, Positive-Sequence)  nominalFrequency=60  samplingRate=24  reportingFactor=1
  PMU_07 : spsPMUPLLBasedPositiveSequenceLib/PMU (PLL-Based, Positive-Sequence)  nominalFrequency=60  samplingRate=24  reportingFactor=1
  PMU_{19..24,68} (7 alike) : spsPMUPLLBasedPositiveSequenceLib/PMU (PLL-Based, Positive-Sequence)  nominalFrequency=60  samplingRate=24  reportingFactor=1
  Scope_F_area1 : Scope
  Scope_V_area1 : Scope
  wires:
  [Vabc_04] -> PMU_04/1
  [Vabc_05] -> PMU_05/1
  [Vabc_06] -> PMU_06/1
  [Vabc_07] -> PMU_07/1
  [Vabc_19] -> PMU_19/1
  [Vabc_20] -> PMU_20/1
  [Vabc_21] -> PMU_21/1
  [Vabc_22] -> PMU_22/1
  [Vabc_23] -> PMU_23/1
  [Vabc_24] -> PMU_24/1
  [Vabc_68] -> PMU_68/1
  PMU_04/1 -> MuxV/1
  PMU_04/3 -> MuxF/1
  PMU_05/1 -> MuxV/2
  PMU_05/3 -> MuxF/2
  PMU_06/1 -> MuxV/3
  PMU_06/3 -> MuxF/3
  PMU_07/1 -> MuxV/4
  PMU_07/3 -> MuxF/4
  PMU_19/1 -> MuxV/5
  PMU_19/3 -> MuxF/5
  PMU_20/1 -> MuxV/6
  PMU_20/3 -> MuxF/6
  PMU_21/1 -> MuxV/7
  PMU_21/3 -> MuxF/7
  PMU_22/1 -> MuxV/8
  PMU_22/3 -> MuxF/8
  PMU_23/1 -> MuxV/9
  PMU_23/3 -> MuxF/9
  PMU_24/1 -> MuxV/10
  PMU_24/3 -> MuxF/10
  PMU_68/1 -> MuxV/11
  PMU_68/3 -> MuxF/11
  MuxV/1 -> Scope_V_area1/1, Log_V_area1/1
  MuxF/1 -> Scope_F_area1/1, Log_F_area1/1

== system IEEE_BUS_68_AGC/PMU Monitoring/area2 ==
  Log_F_area2 : ToWorkspace  VariableName=F_area2  SaveFormat=Structure With Time  SampleTime=0.00833333333333333
  Log_V_area2 : ToWorkspace  VariableName=V_area2  SaveFormat=Structure With Time  SampleTime=0.00833333333333333
  MuxF : Mux  Inputs=16
  MuxV : Mux  Inputs=16
  PMU_02 : spsPMUPLLBasedPositiveSequenceLib/PMU (PLL-Based, Positive-Sequence)  nominalFrequency=60  samplingRate=24  reportingFactor=1
  PMU_03 : spsPMUPLLBasedPositiveSequenceLib/PMU (PLL-Based, Positive-Sequence)  nominalFrequency=60  samplingRate=24  reportingFactor=1
  PMU_{37,52,55..60,62..67} (14 alike) : spsPMUPLLBasedPositiveSequenceLib/PMU (PLL-Based, Positive-Sequence)  nominalFrequency=60  samplingRate=24  reportingFactor=1
  Scope_F_area2 : Scope
  Scope_V_area2 : Scope
  wires:
  [Vabc_02] -> PMU_02/1
  [Vabc_03] -> PMU_03/1
  [Vabc_37] -> PMU_37/1
  [Vabc_52] -> PMU_52/1
  [Vabc_55] -> PMU_55/1
  [Vabc_56] -> PMU_56/1
  [Vabc_57] -> PMU_57/1
  [Vabc_58] -> PMU_58/1
  [Vabc_59] -> PMU_59/1
  [Vabc_60] -> PMU_60/1
  [Vabc_62] -> PMU_62/1
  [Vabc_63] -> PMU_63/1
  [Vabc_64] -> PMU_64/1
  [Vabc_65] -> PMU_65/1
  [Vabc_66] -> PMU_66/1
  [Vabc_67] -> PMU_67/1
  PMU_02/1 -> MuxV/1
  PMU_02/3 -> MuxF/1
  PMU_03/1 -> MuxV/2
  PMU_03/3 -> MuxF/2
  PMU_37/1 -> MuxV/3
  PMU_37/3 -> MuxF/3
  PMU_52/1 -> MuxV/4
  PMU_52/3 -> MuxF/4
  PMU_55/1 -> MuxV/5
  PMU_55/3 -> MuxF/5
  PMU_56/1 -> MuxV/6
  PMU_56/3 -> MuxF/6
  PMU_57/1 -> MuxV/7
  PMU_57/3 -> MuxF/7
  PMU_58/1 -> MuxV/8
  PMU_58/3 -> MuxF/8
  PMU_59/1 -> MuxV/9
  PMU_59/3 -> MuxF/9
  PMU_60/1 -> MuxV/10
  PMU_60/3 -> MuxF/10
  PMU_62/1 -> MuxV/11
  PMU_62/3 -> MuxF/11
  PMU_63/1 -> MuxV/12
  PMU_63/3 -> MuxF/12
  PMU_64/1 -> MuxV/13
  PMU_64/3 -> MuxF/13
  PMU_65/1 -> MuxV/14
  PMU_65/3 -> MuxF/14
  PMU_66/1 -> MuxV/15
  PMU_66/3 -> MuxF/15
  PMU_67/1 -> MuxV/16
  PMU_67/3 -> MuxF/16
  MuxV/1 -> Scope_V_area2/1, Log_V_area2/1
  MuxF/1 -> Scope_F_area2/1, Log_F_area2/1

== system IEEE_BUS_68_AGC/PMU Monitoring/area3 ==
  Log_F_area3 : ToWorkspace  VariableName=F_area3  SaveFormat=Structure With Time  SampleTime=0.00833333333333333
  Log_V_area3 : ToWorkspace  VariableName=V_area3  SaveFormat=Structure With Time  SampleTime=0.00833333333333333
  MuxF : Mux  Inputs=11
  MuxV : Mux  Inputs=11
  PMU_01 : spsPMUPLLBasedPositiveSequenceLib/PMU (PLL-Based, Positive-Sequence)  nominalFrequency=60  samplingRate=24  reportingFactor=1
  PMU_08 : spsPMUPLLBasedPositiveSequenceLib/PMU (PLL-Based, Positive-Sequence)  nominalFrequency=60  samplingRate=24  reportingFactor=1
  PMU_09 : spsPMUPLLBasedPositiveSequenceLib/PMU (PLL-Based, Positive-Sequence)  nominalFrequency=60  samplingRate=24  reportingFactor=1
  PMU_{25..29,47,53..54} (8 alike) : spsPMUPLLBasedPositiveSequenceLib/PMU (PLL-Based, Positive-Sequence)  nominalFrequency=60  samplingRate=24  reportingFactor=1
  Scope_F_area3 : Scope
  Scope_V_area3 : Scope
  wires:
  [Vabc_01] -> PMU_01/1
  [Vabc_08] -> PMU_08/1
  [Vabc_09] -> PMU_09/1
  [Vabc_25] -> PMU_25/1
  [Vabc_26] -> PMU_26/1
  [Vabc_27] -> PMU_27/1
  [Vabc_28] -> PMU_28/1
  [Vabc_29] -> PMU_29/1
  [Vabc_47] -> PMU_47/1
  [Vabc_53] -> PMU_53/1
  [Vabc_54] -> PMU_54/1
  PMU_01/1 -> MuxV/1
  PMU_01/3 -> MuxF/1
  PMU_08/1 -> MuxV/2
  PMU_08/3 -> MuxF/2
  PMU_09/1 -> MuxV/3
  PMU_09/3 -> MuxF/3
  PMU_25/1 -> MuxV/4
  PMU_25/3 -> MuxF/4
  PMU_26/1 -> MuxV/5
  PMU_26/3 -> MuxF/5
  PMU_27/1 -> MuxV/6
  PMU_27/3 -> MuxF/6
  PMU_28/1 -> MuxV/7
  PMU_28/3 -> MuxF/7
  PMU_29/1 -> MuxV/8
  PMU_29/3 -> MuxF/8
  PMU_47/1 -> MuxV/9
  PMU_47/3 -> MuxF/9
  PMU_53/1 -> MuxV/10
  PMU_53/3 -> MuxF/10
  PMU_54/1 -> MuxV/11
  PMU_54/3 -> MuxF/11
  MuxV/1 -> Scope_V_area3/1, Log_V_area3/1
  MuxF/1 -> Scope_F_area3/1, Log_F_area3/1

== system IEEE_BUS_68_AGC/PMU Monitoring/area4 ==
  Log_F_area4_new : ToWorkspace  VariableName=F_area4  SaveFormat=Structure With Time  SampleTime=0.00833333333333333
  Log_V_area4_new : ToWorkspace  VariableName=V_area4  SaveFormat=Structure With Time  SampleTime=0.00833333333333333
  MuxF : Mux  Inputs=22
  MuxV : Mux  Inputs=22
  PMU_{10..13,17,30..36,38..39,43..46,49..51,61} (22 alike) : spsPMUPLLBasedPositiveSequenceLib/PMU (PLL-Based, Positive-Sequence)  nominalFrequency=60  samplingRate=24  reportingFactor=1
  Scope_F_area4_new : Scope
  Scope_V_area4_new : Scope
      settings: ActiveDisplayYMinimum=0.84640534519710031  ActiveDisplayYMaximum=1.1857598592732532
  wires:
  [Vabc_10] -> PMU_10/1
  [Vabc_11] -> PMU_11/1
  [Vabc_12] -> PMU_12/1
  [Vabc_13] -> PMU_13/1
  [Vabc_17] -> PMU_17/1
  [Vabc_30] -> PMU_30/1
  [Vabc_31] -> PMU_31/1
  [Vabc_32] -> PMU_32/1
  [Vabc_33] -> PMU_33/1
  [Vabc_34] -> PMU_34/1
  [Vabc_35] -> PMU_35/1
  [Vabc_36] -> PMU_36/1
  [Vabc_38] -> PMU_38/1
  [Vabc_39] -> PMU_39/1
  [Vabc_43] -> PMU_43/1
  [Vabc_44] -> PMU_44/1
  [Vabc_45] -> PMU_45/1
  [Vabc_46] -> PMU_46/1
  [Vabc_49] -> PMU_49/1
  [Vabc_50] -> PMU_50/1
  [Vabc_51] -> PMU_51/1
  [Vabc_61] -> PMU_61/1
  PMU_10/1 -> MuxV/1
  PMU_10/3 -> MuxF/1
  PMU_11/1 -> MuxV/2
  PMU_11/3 -> MuxF/2
  PMU_12/1 -> MuxV/3
  PMU_12/3 -> MuxF/3
  PMU_13/1 -> MuxV/4
  PMU_13/3 -> MuxF/4
  PMU_17/1 -> MuxV/5
  PMU_17/3 -> MuxF/5
  PMU_30/1 -> MuxV/6
  PMU_30/3 -> MuxF/6
  PMU_31/1 -> MuxV/7
  PMU_31/3 -> MuxF/7
  PMU_32/1 -> MuxV/8
  PMU_32/3 -> MuxF/8
  PMU_33/1 -> MuxV/9
  PMU_33/3 -> MuxF/9
  PMU_34/1 -> MuxV/10
  PMU_34/3 -> MuxF/10
  PMU_35/1 -> MuxV/11
  PMU_35/3 -> MuxF/11
  PMU_36/1 -> MuxV/12
  PMU_36/3 -> MuxF/12
  PMU_38/1 -> MuxV/13
  PMU_38/3 -> MuxF/13
  PMU_39/1 -> MuxV/14
  PMU_39/3 -> MuxF/14
  PMU_43/1 -> MuxV/15
  PMU_43/3 -> MuxF/15
  PMU_44/1 -> MuxV/16
  PMU_44/3 -> MuxF/16
  PMU_45/1 -> MuxV/17
  PMU_45/3 -> MuxF/17
  PMU_46/1 -> MuxV/18
  PMU_46/3 -> MuxF/18
  PMU_49/1 -> MuxV/19
  PMU_49/3 -> MuxF/19
  PMU_50/1 -> MuxV/20
  PMU_50/3 -> MuxF/20
  PMU_51/1 -> MuxV/21
  PMU_51/3 -> MuxF/21
  PMU_61/1 -> MuxV/22
  PMU_61/3 -> MuxF/22
  MuxV/1 -> Scope_V_area4_new/1, Log_V_area4_new/1
  MuxF/1 -> Scope_F_area4_new/1, Log_F_area4_new/1

== system IEEE_BUS_68_AGC/PMU Monitoring/area5 ==
  Log_F_area5 : ToWorkspace  VariableName=F_area5  SaveFormat=Structure With Time  SampleTime=0.00833333333333333
  Log_V_area5 : ToWorkspace  VariableName=V_area5  SaveFormat=Structure With Time  SampleTime=0.00833333333333333
  MuxF : Mux  Inputs=8
  MuxV : Mux  Inputs=8
  PMU_{14..16,18,40..42,48} (8 alike) : spsPMUPLLBasedPositiveSequenceLib/PMU (PLL-Based, Positive-Sequence)  nominalFrequency=60  samplingRate=24  reportingFactor=1
  Scope_F_area5 : Scope
  Scope_V_area5 : Scope
      settings: ActiveDisplayYMinimum=0.97994290518380289  ActiveDisplayYMaximum=1.1000452693526483
  wires:
  [Vabc_14] -> PMU_14/1
  [Vabc_15] -> PMU_15/1
  [Vabc_16] -> PMU_16/1
  [Vabc_18] -> PMU_18/1
  [Vabc_40] -> PMU_40/1
  [Vabc_41] -> PMU_41/1
  [Vabc_42] -> PMU_42/1
  [Vabc_48] -> PMU_48/1
  PMU_14/1 -> MuxV/1
  PMU_14/3 -> MuxF/1
  PMU_15/1 -> MuxV/2
  PMU_15/3 -> MuxF/2
  PMU_16/1 -> MuxV/3
  PMU_16/3 -> MuxF/3
  PMU_18/1 -> MuxV/4
  PMU_18/3 -> MuxF/4
  PMU_40/1 -> MuxV/5
  PMU_40/3 -> MuxF/5
  PMU_41/1 -> MuxV/6
  PMU_41/3 -> MuxF/6
  PMU_42/1 -> MuxV/7
  PMU_42/3 -> MuxF/7
  PMU_48/1 -> MuxV/8
  PMU_48/3 -> MuxF/8
  MuxV/1 -> Scope_V_area5/1, Log_V_area5/1
  MuxF/1 -> Scope_F_area5/1, Log_F_area5/1

== system IEEE_BUS_68_AGC/area-1/Automatic Generation Control without economic dispatch process2 ==
  dw : Inport
  AGC Status : Inport  Port=2
  AGC Switch : Switch  Criteria=u2 > Threshold  SaturateOnIntegerOverflow=off  InputSameDT=off
  Area control frequency error to PI controller : slpidlib/PID Controller (2DOF)  Controller=PI  Form=Parallel  TimeDomain=Continuous-time  UseExternalTs=off  SampleTime=1  IntegratorMethod=Forward Euler  FilterMethod=Forward Euler  ControllerParametersSource=internal  P=0.75  I=2.5  UseKiTs=off  D=0  UseExternalDerivativeSource=off  N=100  UseFilter=on  b=1  c=1  TunerSelectOption=Transfer Function Based (PID Tuner App)  InitialConditionSource=internal  InitialConditionForIntegrator=0  InitialConditionForFilter=0  DifferentiatorICPrevScaledInput=0  ExternalReset=none  TrackingMode=off  Kt=1  LimitOutput=off  SatLimitsSource=internal  UpperSaturationLimit=inf  LowerSaturationLimit=-inf  LinearizeAsGain=on  AntiWindupMode=none  Kb=1  LimitIntegrator=off  UpperIntegratorSaturationLimit=inf  LowerIntegratorSaturationLimit=-inf  POutMin=[]  POutMax=[]  IOutMin=[]  IOutMax=[]  DOutMin=[]  DOutMax=[]  NOutMin=[]  NOutMax=[]  bOutMin=[]  bOutMax=[]  cOutMin=[]  cOutMax=[]  SumOutMin=[]  SumOutMax=[]  SaturationOutMin=[]  SaturationOutMax=[]  PParamMin=[]  PParamMax=[]  IParamMin=[]  IParamMax=[]  DParamMin=[]  DParamMax=[]  NParamMin=[]  NParamMax=[]  bParamMin=[]  bParamMax=[]  cParamMin=[]  cParamMax=[]  KbParamMin=[]  KbParamMax=[]  KtParamMin=[]  KtParamMax=[]  KbOutMin=[]  KbOutMax=[]  KtOutMin=[]  KtOutMax=[]  IntegratorOutMin=[]  IntegratorOutMax=[]  FilterOutMin=[]  FilterOutMax=[]  SumI1OutMin=[]  SumI1OutMax=[]  SumI2OutMin=[]  SumI2OutMax=[]  SumI3OutMin=[]  SumI3OutMax=[]  SumI4OutMin=[]  SumI4OutMax=[]  SumDOutMin=[]  SumDOutMax=[]  Sum1OutMin=[]  Sum1OutMax=[]  Sum2OutMin=[]  Sum2OutMax=[]  Sum3OutMin=[]  Sum3OutMax=[]  DifferentiatorOutMin=[]  DifferentiatorOutMax=[]  FilterDiffOutCoefMin=[]  FilterDiffOutCoefMax=[]  ReciprocalOutMin=[]  ReciprocalOutMax=[]  SumDenOutMin=[]  SumDenOutMax=[]  SumNumOutMin=[]  SumNumOutMax=[]  DivideOutMin=[]  DivideOutMax=[]  UdiffTsProdOutMin=[]  UdiffTsProdOutMax=[]  NTsProdOutMin=[]  NTsProdOutMax=[]  UintegralTsProdOutMin=[]  UintegralTsProdOutMax=[]  UngainTsProdOutMin=[]  UngainTsProdOutMax=[]  ClampingZeroOutDataTypeStr=Inherit: Inherit via back propagation  ClampingZeroOutMin=[]  ClampingZeroOutMax=[]  FilterDenConstantOutDataTypeStr=Inherit: Inherit via back propagation  FilterDenConstantOutMin=[]  FilterDenConstantOutMax=[]  PCopyOutDataTypeStr=Inherit: Inherit via back propagation  PCopyOutMin=[]  PCopyOutMax=[]  NCopyOutDataTypeStr=Inherit: Inherit via back propagation  NCopyOutMin=[]  NCopyOutMax=[]  IntegratorContinuousStateAttributes=''  IntegratorStateMustResolveToSignalObject=off  IntegratorRTWStateStorageClass=Auto  FilterContinuousStateAttributes=''  FilterStateMustResolveToSignalObject=off  FilterRTWStateStorageClass=Auto  ParallelPVariant=InternalParameters  IdealPVariant=Disabled  IVariant=InternalParameters  DVariant=Disabled  bVariant=InternalParameters  cVariant=Disabled  IntegratorVariant=Continuous  SatVariant=Disabled  AWVariant=Passthrough  PCopyVariant=Disabled  TRVariant=Disabled  FdbkBlocksVariant=Forward  IdealPFdbkVariant=Disabled  SatFdbkVariant=Disabled  DerivativeFilterVariant=Disabled  NVariant=Disabled  NCopyVariant=Disabled_SignalSpec  FilterICVariant=Disabled  IntegratorICVariant=InternalICs  ExternalResetVariant=Disabled  TRSumVariant=Passthrough  SumFdbkVariant=Disabled  SumVariant=Sum_PI  TsampFilterVariant=InternalTs  TsampNgainVariant=Passthrough  TsampIntegralVariant=Disabled_SignalSpec  ExternalSaturationOutDataTypeStr=Inherit: Same as second input  DerivativeSourceVariant=Disabled  PreIntVariant=InternalPreInt
  Zero deviation : Constant  Value=0
  Delta_P : Outport
  wires:
  Area control frequency error to PI controller/1 -> Delta_P/1
  AGC Switch/1 -> Area control frequency error to PI controller/2
  Zero deviation/1 -> AGC Switch/3, Area control frequency error to PI controller/1
  dw/1 -> AGC Switch/1
  AGC Status/1 -> AGC Switch/2

== system IEEE_BUS_68_AGC/area-1/gen4 ==
  "M4: Turbine & Regulators " : Subsystem
  Synchronous Machine SI Fundamental : spsSynchronousMachineSIFundamentalLib/Synchronous Machine SI Fundamental  Commented=on  PresetModel=No  MechanicalLoad=Mechanical power Pm  ShowDetailedParameters=on  RotorType=Salient-pole  Units=SI fundamental parameters  MeasurementBus=off  NominalParameters="[ 187E6  13800   60   1087 ]"  Stator="[ 2.9069E-03  3.0892E-04  3.2164E-03  9.7153E-04 ]"  Field="[ 5.9013E-04  3.0712E-04 ]"  Dampers2=[ 0.0664, 1.387e-3, 0.0292, 6.896e-4, 7.907e-3, 2.477e-3]  Dampers1="[ 1.1900E-02  4.9076E-04  2.0081E-02  1.0365E-03 ]"  Mechanical=[ 3.895e6 0 20 ]  PolePairs=20  InitialConditions="[ 0  0  0  0  0  0  0  0  70.3192 ]"  SetSaturation=off  Saturation=[695.64,774.7,917.5,1001.6,1082.2,1175.9,1293.6,1430.2,1583.7;9660,10623,12243,13063,13757,14437,15180,15890,16567]  DisplayVfd=off  LoadFlowParameters=[1,0,0,0,0]  TsPowergui=0  TsBlock=-1  IterativeModel=Trapezoidal non iterative  IterativeDiscreteModel=Trapezoidal non iterative  BusType=PV  Pref=0  Qref=0  Qmin=-inf  Qmax=inf  PLF=0  QLF=0
      settings: LibrarySourceBlock=|
      | sps_lib/Electrical Machines/Synchronous Machine
      | SI Fundamental
  Synchronous Machine pu Standard : spsSynchronousMachinepuStandardLib/Synchronous Machine pu Standard  Commented=on  PresetModel=No  MechanicalLoad=Mechanical power Pm  ShowDetailedParameters=on  RotorType=Salient-pole  Units=per unit standard parameters  MeasurementBus=off  NominalParameters=[6e+04 400 50]  Reactances1=[ 1.81, 0.3, 0.23, 1.76, 0.65, 0.25, 0.15 ]  Reactances2=[2.24 0.17 0.12 1.02 0.13 0.08]  dAxisTimeConstants=Short-circuit  qAxisTimeConstants=Short-circuit  TimeConstants1="[ 4.4849  0.0681  0.1  ]"  TimeConstants2=[ 8.0, 0.03, 1.0, 0.07 ]  TimeConstants3="[  4.49  0.0681  0.0513  ]"  TimeConstants4=[ 8.0, 0.03, 0.3371, 0.0295 ]  TimeConstants5=[ 1.01, 0.053, 0.1 ]  TimeConstants6=[ 1.3201, 0.023, 1.0, 0.07 ]  TimeConstants7=[0.012 0.003 0.003]  TimeConstants8=[ 1.3201, 0.0231, 0.3371, 0.0295 ]  StatorResistance=0.037875  Mechanical=[0.1028 0.02056 2]  PolePairs=20  InitialConditions="[ 0  0  0  0  0  0  0  0  1 ]"  SetSaturation=on  Saturation=[0.6404,0.7127,0.8441,0.9214,0.9956,1.082,1.19,1.316,1.457;0.7,0.7698,0.8872,0.9466,0.9969,1.046,1.1,1.151,1.201]  LoadFlowParameters=[1,0,0,0,0]  TsPowergui=0  TsBlock=-1  IterativeModel=Trapezoidal non iterative  IterativeDiscreteModel=Trapezoidal non iterative  BusType=PV  Pref=0  Qref=0  Qmin=-inf  Qmax=inf  PLF=0  QLF=0
  Vref4 : Constant  Value=0.997
  gen4 : spsSynchronousMachinepuStandardLib/Synchronous Machine pu Standard  PresetModel=No  MechanicalLoad=Mechanical power Pm  ShowDetailedParameters=on  RotorType=Round  Units=per unit standard parameters  MeasurementBus=off  NominalParameters="[1000*1e6  13.8*1e3   60 ]"  Reactances1="[mac_con(4,6:8)  mac_con(4,11:13)  mac_con(4,4)]"  Reactances2=[ 1.305, 0.296, 0.252, 0.474, 0.243, 0.18 ]  dAxisTimeConstants=Open-circuit  qAxisTimeConstants=Open-circuit  TimeConstants1=[]  TimeConstants2="[mac_con(4,9:10)  mac_con(4,14:15)]"  TimeConstants3=[]  TimeConstants4=[]  TimeConstants5=[ 1.01, 0.053, 0.1 ]  TimeConstants6=[]  TimeConstants7=[]  TimeConstants8=[]  StatorResistance=mac_con(4,5)  Mechanical="[ mac_con(4,16)  0  4]"  PolePairs=4  InitialConditions=[0 -81.725 0.63416 0.63416 0.63416 0.5523 -119.448 120.552 1.00606]  SetSaturation=off  Saturation=[0.6404,0.7127,0.8441,0.9214,0.9956,1.082,1.19,1.316,1.457;0.7,0.7698,0.8872,0.9466,0.9969,1.046,1.1,1.151,1.201]  LoadFlowParameters=[1 830000000 0 0 0]  TsPowergui=0  TsBlock=-1  IterativeModel=Trapezoidal non iterative  IterativeDiscreteModel=Trapezoidal non iterative  BusType=PV  Pref=632000000  Qref=0  Qmin=-Inf  Qmax=Inf  PLF=0  QLF=0
  A : PMIOPort  Side=Left
  B : PMIOPort  Port=2  Side=Left
  C : PMIOPort  Port=3  Side=Left
  wires:
  "M4: Turbine & Regulators "/1(Pm4) -> gen4/1
  "M4: Turbine & Regulators "/2(Vf4) -> gen4/2
  gen4/1 -> "M4: Turbine & Regulators "/1(m4)
  [PSSmodel] -> "M4: Turbine & Regulators "/4(PSS4)
  Vref4/1 -> "M4: Turbine & Regulators "/3(Vref4)
  [Pref_G4] -> "M4: Turbine & Regulators "/2(Pref4)
  connections:
  A/RConn1 -- gen4/RConn1
  B/RConn1 -- gen4/RConn2
  C/RConn1 -- gen4/RConn3
